simulink model "FMT_ExtINS_DataSIM"  (R2026b)
settings: Solver=FixedStepDiscrete  StopTime=26  FixedStep=0.0005
settings Model: Creator=26718  LastModifiedBy=26718
settings DataIOCC: ExternalInput=fmt_default_input('FMT_ExtINS_DataSIM')  LoadExternalInput=on
settings DebuggingCC: AlgebraicLoopMsg=error

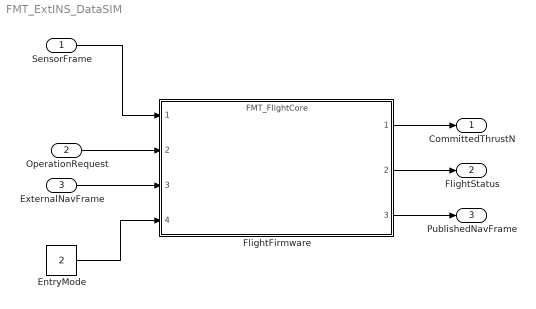
== system FMT_ExtINS_DataSIM ==
  SensorFrame : Inport  OutDataTypeStr=double  PortDimensions=18  SampleTime=0.0005  Interpolate=off
  OperationRequest : Inport  Port=2  OutDataTypeStr=double  PortDimensions=2  SampleTime=0.0005  Interpolate=off
  ExternalNavFrame : Inport  Port=3  OutDataTypeStr=uint8  PortDimensions=fmt_flight_nav_width  SampleTime=0.0005  Interpolate=off
  EntryMode : Constant  Value=2
  FlightFirmware : ModelReference  ModelNameDialog=FMT_FlightCore  SimulationMode=Normal  ModelReferenceVersion=1.1
  CommittedThrustN : Outport
  FlightStatus : Outport  Port=2
  PublishedNavFrame : Outport  Port=3
  wires:
  OperationRequest/1 -> FlightFirmware/2
  ExternalNavFrame/1 -> FlightFirmware/3
  SensorFrame/1 -> FlightFirmware/1
  FlightFirmware/3 -> PublishedNavFrame/1
  FlightFirmware/2 -> FlightStatus/1
  FlightFirmware/1 -> CommittedThrustN/1
  EntryMode/1 -> FlightFirmware/4
